simulink model "Plant"  (R2018b)
settings: configuration reference "plant_config" (kept outside this file)
values from neighbouring files (symbols this model uses):
  PLANT_EXPORT = Simulink.Parameter(PLANT_EXPORT_VALUE)    [plant_model_init.m]
  PLANT_PARAM = Simulink.Parameter(PLANT_PARAM_VALUE)    [plant_model_init.m]
undefined symbols (not defined in the file or in its folder): acc_x, acc_x_O, acc_y, acc_y_O, acc_z, acc_z_O, alt, alt_0, day, DiscIntNeverNeededParam, fixType, flags, gSpeed, gyr_x, gyr_y, gyr_z, h_R, hAcc, heading, headingAcc, height, hMSL, hour, iTOW, lat, lon, M_BO, M_OB, mag_x, mag_y, mag_z, month, nano, numSV, pDOP, phi, PLANT_CONST, plant_model, pressure, prop_vel, psi, quat, reserved1, reserved2, rot_x_B, rot_y_B, rot_z_B, sAcc, sec, Sensor_Model, tAcc, temperature, temprature, theta, timestamp, vAcc, valid, vel_x_O, vel_y_O, vel_z_O ... (+6)
libraries: FMT_Model_Lib x13, dspsrcs4 x6, simulink x4, aerolibatmos2 x1
(part 1 of 2)
settings Model: Creator=jc  LastModifiedBy=zouji
settings ConfigSetRef: SourceLocation=Base Workspace

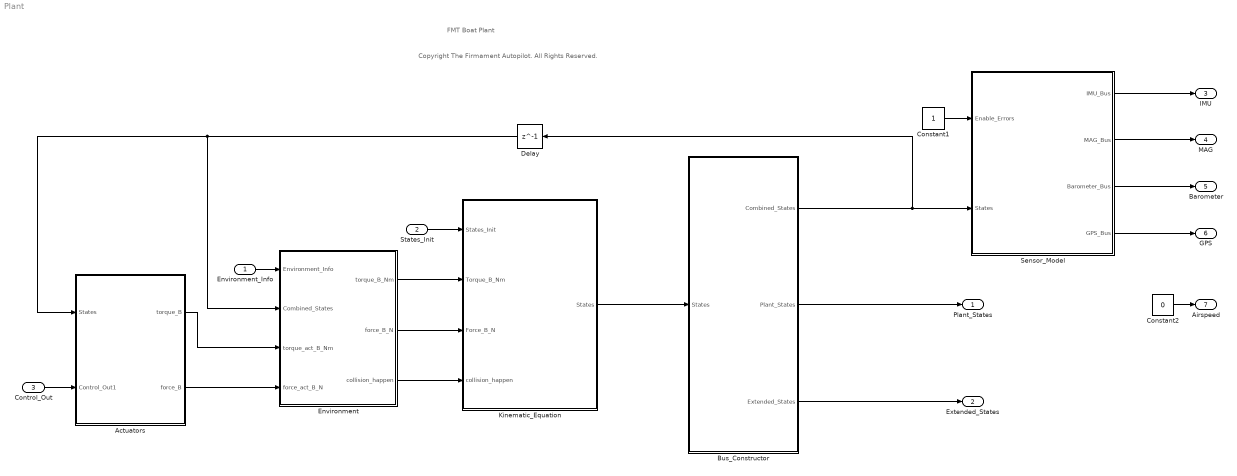
== system Plant ==
  note: FMT Boat Plant
  note: Copyright The Firmament Autopilot. All Rights Reserved.
  Environment_Info : Inport  OutDataTypeStr=Bus: Environment_Info_Bus  Interpolate=off
  States_Init : Inport  Port=2  OutDataTypeStr=Bus: States_Init_Bus  Interpolate=off
  Control_Out : Inport  Port=3  OutDataTypeStr=Bus: Control_Out_Bus  Interpolate=off
  Actuators : Subsystem  TreatAsAtomicUnit=on
  Bus_Constructor : Subsystem  TreatAsAtomicUnit=on  mask{lat_0=PLANT_PARAM.LAT_0, lon_0=PLANT_PARAM.LON_0, hgt_0=PLANT_PARAM.ALT_0}
      mask prompts: lat_0 "init latitude (rad)"; lon_0 "init lontitude (rad)"; hgt_0 "init height (m)"
  Constant1 : Constant  OutDataTypeStr=Inherit: Inherit via back propagation
  Constant2 : Constant  Value=0  OutDataTypeStr=Bus: AirSpeed_Bus
  Delay : Delay  DelayLength=1
  Environment : Subsystem  TreatAsAtomicUnit=on
  Kinematic_Equation : Subsystem  TreatAsAtomicUnit=on
  Sensor_Model : Subsystem  TreatAsAtomicUnit=on
  Plant_States : Outport  OutDataTypeStr=Bus: Plant_States_Bus
  Extended_States : Outport  Port=2  OutDataTypeStr=Bus: Extended_States_Bus
  IMU : Outport  Port=3  OutDataTypeStr=Bus: IMU_Bus
  MAG : Outport  Port=4  OutDataTypeStr=Bus: MAG_Bus
  Barometer : Outport  Port=5  OutDataTypeStr=Bus: Barometer_Bus
  GPS : Outport  Port=6  OutDataTypeStr=Bus: GPS_uBlox_Bus
  Airspeed : Outport  Port=7  OutDataTypeStr=Bus: AirSpeed_Bus
  wires:
  Kinematic_Equation/1(States) -> Bus_Constructor/1(States)
  Control_Out/1 -> Actuators/2(Control_Out1)
  Constant1/1 -> Sensor_Model/1(Enable_Errors)
  Sensor_Model/1(IMU_Bus) -> IMU/1
  Sensor_Model/2(MAG_Bus) -> MAG/1
  Sensor_Model/3(Barometer_Bus) -> Barometer/1
  Sensor_Model/4(GPS_Bus) -> GPS/1
  Bus_Constructor/3(Extended_States) -> Extended_States/1
  Bus_Constructor/1(Combined_States) -> Sensor_Model/2(States), Delay/1
  Constant2/1 -> Airspeed/1
  Bus_Constructor/2(Plant_States) -> Plant_States/1
  Delay/1 -> Environment/2(Combined_States), Actuators/1(States)
  Environment/3(collision_happen) -> Kinematic_Equation/4(collision_happen)
  States_Init/1 -> Kinematic_Equation/1(States_Init)
  Actuators/2(force_B) -> Environment/4(force_act_B_N)
  Actuators/1(torque_B) -> Environment/3(torque_act_B_Nm)
  Environment_Info/1 -> Environment/1(Environment_Info)
  Environment/1(torque_B_Nm) -> Kinematic_Equation/2(Torque_B_Nm)
  Environment/2(force_B_N) -> Kinematic_Equation/3(Force_B_N)

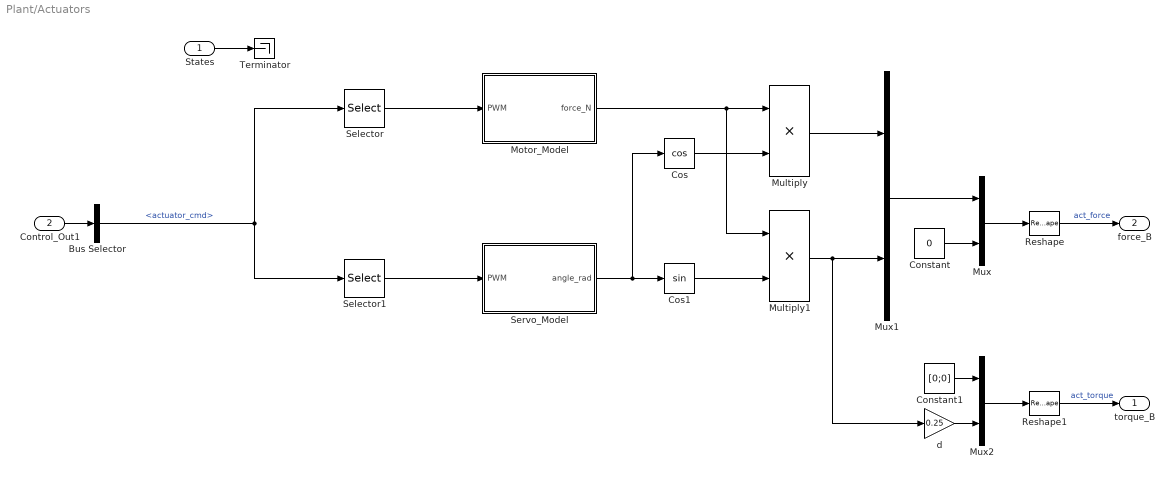
== system Plant/Actuators ==
  States : Inport
  Control_Out1 : Inport  Port=2
  Bus Selector : BusSelector  OutputSignals=actuator_cmd
  Constant : Constant  Value=0  OutDataTypeStr=single
  Constant1 : Constant  Value=[0;0]  VectorParams1D=off  OutDataTypeStr=single
  Cos : Trigonometry  Operator=cos
  Cos1 : Trigonometry
  Motor_Model : Subsystem
  Multiply : Product
  Multiply1 : Product
  Mux : Mux  Inputs=2
  Mux1 : Mux  Inputs=2
  Mux2 : Mux  Inputs=2
  Reshape : Reshape  OutputDimensionality=Column vector (2-D)
  Reshape1 : Reshape  OutputDimensionality=Column vector (2-D)
  Selector : Selector  InputPortWidth=16  IndexOptions=Index vector (dialog)  Indices=1  OutputSizes=1
  Selector1 : Selector  InputPortWidth=16  IndexOptions=Index vector (dialog)  Indices=2  OutputSizes=1
  Servo_Model : Subsystem
  Terminator : Terminator
  d : Gain  Gain=0.25
  torque_B : Outport
  force_B : Outport  Port=2
  wires:
  Control_Out1/1 -> Bus Selector/1
  States/1 -> Terminator/1
  Selector/1 -> Motor_Model/1(PWM)
  Selector1/1 -> Servo_Model/1(PWM)
  Bus Selector/1 -> Selector1/1, Selector/1  "<actuator_cmd>"
  Servo_Model/1(angle_rad) -> Cos1/1, Cos/1
  Cos/1 -> Multiply/2
  Motor_Model/1(force_N) -> Multiply1/1, Multiply/1
  Cos1/1 -> Multiply1/2
  Multiply/1 -> Mux1/1
  Constant/1 -> Mux/2
  Mux1/1 -> Mux/1
  Mux/1 -> Reshape/1
  Reshape/1 -> force_B/1  "act_force"
  Multiply1/1 -> d/1, Mux1/2
  Mux2/1 -> Reshape1/1
  Reshape1/1 -> torque_B/1  "act_torque"
  Constant1/1 -> Mux2/1
  d/1 -> Mux2/2

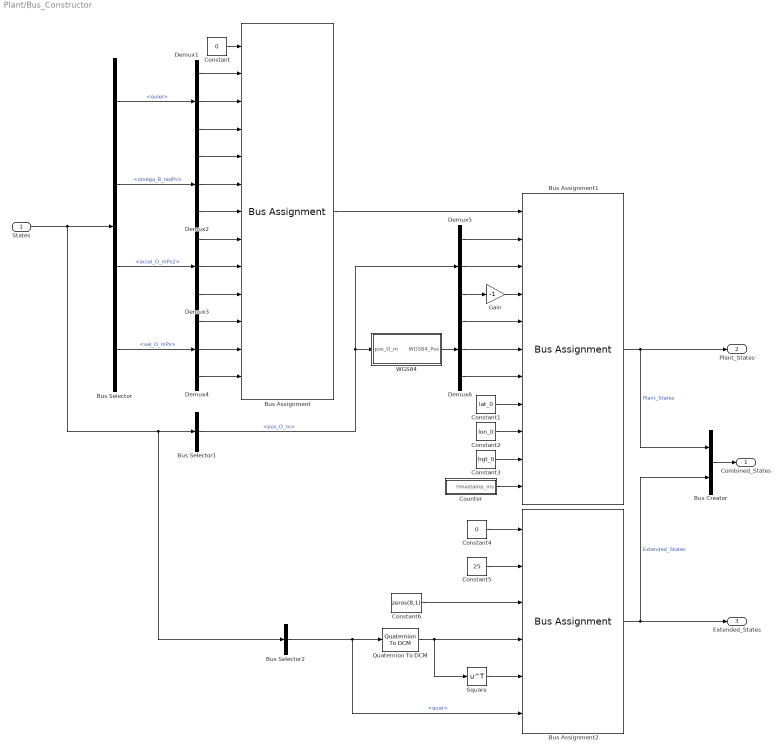
== system Plant/Bus_Constructor ==
  States : Inport
  Bus Assignment : BusAssignment  AssignedSignals=phi,theta,psi,rot_x_B,rot_y_B,rot_z_B,acc_x_O,acc_y_O,acc_z_O,vel_x_O,vel_y_O,vel_z_O
  Bus Assignment1 : BusAssignment  AssignedSignals=x_R,y_R,h_R,lat,lon,alt,lat_0,lon_0,alt_0,timestamp
  Bus Assignment2 : BusAssignment  AssignedSignals=temprature,prop_vel,M_BO,M_OB,quat
  Bus Creator : BusCreator  Inputs=2
  Bus Selector : BusSelector  OutputSignals=euler,omega_B_radPs,accel_O_mPs2,vel_O_mPs
  Bus Selector1 : BusSelector  OutputSignals=pos_O_m
  Bus Selector2 : BusSelector  OutputSignals=quat
  Constant : Constant  Value=0  OutDataTypeStr=Bus: Plant_States_Bus
  Constant1 : Constant  Value=lat_0
  Constant2 : Constant  Value=lon_0
  Constant3 : Constant  Value=hgt_0
  Constant4 : Constant  Value=0  OutDataTypeStr=Bus: Extended_States_Bus
  Constant5 : Constant  Value=25  OutDataTypeStr=Inherit: Inherit via back propagation
  Constant6 : Constant  Value=zeros(8,1)  OutDataTypeStr=single
  Counter : Subsystem
  Demux{1..6} (6 alike) : Demux  Outputs=3
  Gain : Gain  Gain=-1  OutDataTypeStr=Inherit: Same as input
  Quaternion To DCM : FMT_Model_Lib/Quaternion/Quaternion To DCM
      settings: SourceProductName=FMT Toolbox
  Square : Math  Operator=transpose  SaturateOnIntegerOverflow=on
  WGS84 : Subsystem
  Combined_States : Outport
  Plant_States : Outport  Port=2
  Extended_States : Outport  Port=3
  wires:
  Constant/1 -> Bus Assignment/1
  States/1 -> Bus Selector2/1, Bus Selector1/1, Bus Selector/1
  Bus Selector/1 -> Demux1/1  "<euler>"
  Bus Selector/2 -> Demux2/1  "<omega_B_radPs>"
  Bus Selector/3 -> Demux3/1  "<accel_O_mPs2>"
  Bus Selector/4 -> Demux4/1  "<vel_O_mPs>"
  Bus Assignment/1 -> Bus Assignment1/1
  Bus Selector1/1 -> Demux5/1, WGS84/1(pos_O_m)  "<pos_O_m>"
  Bus Assignment1/1 -> Plant_States/1, Bus Creator/1  "Plant_States"
  Demux1/2 -> Bus Assignment/3
  Demux5/3 -> Gain/1
  WGS84/1(WGS84_Pos) -> Demux6/1
  Demux1/1 -> Bus Assignment/2
  Demux1/3 -> Bus Assignment/4
  Demux2/1 -> Bus Assignment/5
  Demux2/2 -> Bus Assignment/6
  Demux2/3 -> Bus Assignment/7
  Demux3/1 -> Bus Assignment/8
  Demux3/2 -> Bus Assignment/9
  Demux3/3 -> Bus Assignment/10
  Demux4/1 -> Bus Assignment/11
  Demux4/2 -> Bus Assignment/12
  Demux4/3 -> Bus Assignment/13
  Demux5/2 -> Bus Assignment1/3
  Gain/1 -> Bus Assignment1/4
  Demux5/1 -> Bus Assignment1/2
  Demux6/1 -> Bus Assignment1/5
  Demux6/2 -> Bus Assignment1/6
  Demux6/3 -> Bus Assignment1/7
  Constant2/1 -> Bus Assignment1/9
  Constant1/1 -> Bus Assignment1/8
  Constant3/1 -> Bus Assignment1/10
  Constant4/1 -> Bus Assignment2/1
  Constant5/1 -> Bus Assignment2/2
  Constant6/1 -> Bus Assignment2/3
  Bus Selector2/1 -> Quaternion To DCM/1, Bus Assignment2/6  "<quat>"
  Bus Assignment2/1 -> Bus Creator/2, Extended_States/1  "Extended_States"
  Bus Creator/1 -> Combined_States/1
  Counter/1(timestamp_ms) -> Bus Assignment1/11
  Square/1 -> Bus Assignment2/5
  Quaternion To DCM/1 -> Square/1, Bus Assignment2/4

== system Plant/Environment ==
  Environment_Info : Inport
  Combined_States : Inport  Port=2
  torque_act_B_Nm : Inport  Port=3
  force_act_B_N : Inport  Port=4
  Constant : Constant  Value=0  OutDataTypeStr=Inherit: Inherit via back propagation
  Sum : Sum  Inputs=|++
  Sum1 : Sum  Inputs=|++
  Terminator : Terminator
  Water_Drag : Subsystem  mask{xu=1, xuu=0.5, yv=10, yvv=5, nr=4, nrr=1, mass=plant_model.mass, izz=plant_model.Jzz}
  torque_B_Nm : Outport
  force_B_N : Outport  Port=2
  collision_happen : Outport  Port=3
  wires:
  Environment_Info/1 -> Terminator/1
  Constant/1 -> collision_happen/1
  Combined_States/1 -> Water_Drag/1(Combined_States)
  Water_Drag/1(torque_B_Nm) -> Sum/1  "water_torque"
  Sum/1 -> torque_B_Nm/1  "torque_B_Nm"
  torque_act_B_Nm/1 -> Sum/2
  Water_Drag/2(force_B_N) -> Sum1/1  "water_force"
  force_act_B_N/1 -> Sum1/2
  Sum1/1 -> force_B_N/1  "force_B_N"

== system Plant/Kinematic_Equation ==
  States_Init : Inport
  Torque_B_Nm : Inport  Port=2
  Force_B_N : Inport  Port=3
  collision_happen : Inport  Port=4
  Attitude_Dynamic : Subsystem  mask{Ixx=plant_model.Jxx, Iyy=plant_model.Jyy, Izz=plant_model.Jzz}
  Bus Creator : BusCreator  Inputs=7
  Constant : Constant  Value=0  OutDataTypeStr=Inherit: Inherit via back propagation
  Position_Dynamic : Subsystem  mask{mass=plant_model.mass}
  States : Outport
  wires:
  Attitude_Dynamic/2(omega_B_radPs) -> Position_Dynamic/2(omega_B_radPs), Bus Creator/2  "omega_B_radPs"
  Attitude_Dynamic/3(quat) -> Position_Dynamic/3(quat), Bus Creator/3  "quat"
  collision_happen/1 -> Position_Dynamic/4(vel_reset)
  Bus Creator/1 -> States/1  "states"
  Attitude_Dynamic/1(dot_omega_B_radPs2) -> Bus Creator/1  "dot_omega_B_radPs2"
  Attitude_Dynamic/4(euler) -> Bus Creator/4  "euler"
  Position_Dynamic/1(accel_O_mPs2) -> Bus Creator/5  "accel_O_mPs2"
  Position_Dynamic/2(vel_O_mPs) -> Bus Creator/6  "vel_O_mPs"
  Position_Dynamic/3(pos_O_m) -> Bus Creator/7  "pos_O_m"
  Force_B_N/1 -> Position_Dynamic/1(force_B_N)
  Torque_B_Nm/1 -> Attitude_Dynamic/1(torque_B_Nm)
  Constant/1 -> Attitude_Dynamic/2(rate_reset)
  States_Init/1 -> Position_Dynamic/5(States_Init), Attitude_Dynamic/3(States_Init)

== system Plant/Sensor_Model ==
  Enable_Errors : Inport  OutDataTypeStr=uint8
  States : Inport  Port=2
  Counter : Subsystem
  Sensor_Barometer : Subsystem  TreatAsAtomicUnit=on
  Sensor_GPS : Subsystem  TreatAsAtomicUnit=on
  Sensor_IMU : Subsystem  TreatAsAtomicUnit=on
  Sensor_MAG : Subsystem  TreatAsAtomicUnit=on
  IMU_Bus : Outport
  MAG_Bus : Outport  Port=2
  Barometer_Bus : Outport  Port=3
  GPS_Bus : Outport  Port=4
  wires:
  Counter/1(timestamp_ms) -> Sensor_Barometer/3(timestamp_ms), Sensor_MAG/3(timestamp_ms), Sensor_IMU/3(timestamp_ms), Sensor_GPS/3(timestamp_ms)
  States/1 -> Sensor_GPS/1(States), Sensor_Barometer/1(States), Sensor_MAG/1(States), Sensor_IMU/1(States)
  Sensor_Barometer/1(Barometer_Bus) -> Barometer_Bus/1
  Sensor_MAG/1(MAG_Bus) -> MAG_Bus/1
  Sensor_IMU/1(IMU_Bus) -> IMU_Bus/1
  Enable_Errors/1 -> Sensor_IMU/2(Enable_Errors), Sensor_GPS/2(Enable_Errors), Sensor_Barometer/2(Enable_Errors), Sensor_MAG/2(Enable_Errors)
  Sensor_GPS/1(GPS_Bus) -> GPS_Bus/1

== system Plant/Actuators/Motor_Model ==
  PWM : Inport
  Bias : Bias  Bias=-60.6
  Dead Zone : DeadZone  LowerValue=-1  UpperValue=1  SaturateOnIntegerOverflow=on
  Gain : Gain  Gain=0.0404  OutDataTypeStr=single
  force_N : Outport
  wires:
  Gain/1 -> Bias/1
  Dead Zone/1 -> force_N/1
  PWM/1 -> Gain/1
  Bias/1 -> Dead Zone/1

== system Plant/Actuators/Servo_Model ==
  PWM : Inport
  Bias : Bias  Bias=-270
  Dead Zone : DeadZone  LowerValue=-2  UpperValue=2  SaturateOnIntegerOverflow=on
  Deg2Rad : Gain  Gain=pi/180
  Gain : Gain  Gain=0.18  OutDataTypeStr=single
  Saturation : Saturate  UpperLimit=90  LowerLimit=-90
  angle_rad : Outport
  wires:
  PWM/1 -> Gain/1
  Bias/1 -> Dead Zone/1
  Gain/1 -> Bias/1
  Deg2Rad/1 -> angle_rad/1
  Dead Zone/1 -> Saturation/1
  Saturation/1 -> Deg2Rad/1

== system Plant/Bus_Constructor/Counter ==
  Data Type Conversion2 : DataTypeConversion  OutDataTypeStr=uint32
  Delay : Delay  DelayLength=1  InitialCondition=0
  Sum : Sum  Inputs=|++
  dt : Constant  Value=PLANT_EXPORT.period  OutDataTypeStr=uint32
  timestamp_ms : Outport
  wires:
  dt/1 -> Sum/1
  Sum/1 -> Delay/1
  Delay/1 -> Data Type Conversion2/1
  Data Type Conversion2/1 -> timestamp_ms/1, Sum/2

== system Plant/Bus_Constructor/WGS84 ==
  pos_O_m : Inport
  Add : Sum
  Constant1 : Constant  Value=lat_0
  Constant2 : Constant  Value=lon_0
  Constant3 : Constant  Value=hgt_0
  Data Type Conversion : DataTypeConversion  OutDataTypeStr=double
  Delay : Delay  DelayLength=1
  Delay1 : Delay  DelayLength=1  InitialConditionSource=Input port  InitialCondition=[lat_0;lon_0;hgt_0]
      settings: InputPortMap=u0,p4
  Demux : Demux  Outputs=3
  Divide : Product  Inputs=/*
  Mux : Mux  Inputs=3
  Mux1 : Mux  Inputs=3
  Subtract : Sum  Inputs=+-
  Terminator : Terminator
  WGS84_Derivative : Subsystem
  Zero_Value_Exclusion : Subsystem
  WGS84_Pos : Outport
  wires:
  pos_O_m/1 -> Data Type Conversion/1
  Delay/1 -> Subtract/2
  WGS84_Derivative/1(dx_dlat) -> Mux/1
  Mux/1 -> Zero_Value_Exclusion/1(u)
  Zero_Value_Exclusion/1(y) -> Divide/1
  WGS84_Derivative/3(dz_dh) -> Mux/3
  WGS84_Derivative/2(dy_dlon) -> Mux/2
  Subtract/1 -> Divide/2
  Divide/1 -> Add/1
  Delay1/1 -> Add/2, Demux/1
  Add/1 -> Delay1/1, WGS84_Pos/1
  Demux/1 -> WGS84_Derivative/1(lat_0)
  Demux/3 -> WGS84_Derivative/2(h_0)
  Demux/2 -> Terminator/1
  Data Type Conversion/1 -> Delay/1, Subtract/1
  Mux1/1 -> Delay1/2
  Constant2/1 -> Mux1/2
  Constant1/1 -> Mux1/1
  Constant3/1 -> Mux1/3

== system Plant/Environment/Water_Drag ==
  Combined_States : Inport
  Bus Selector : BusSelector  OutputSignals=Extended_States.M_BO,Plant_States.vel_x_O,Plant_States.vel_y_O,Plant_States.vel_z_O
  Bus Selector1 : BusSelector  OutputSignals=Plant_States.rot_z_B
  Multiply : Product  Multiplication=Matrix(*)
  Mux : Mux  Inputs=3
  Water_Force : Subsystem
  Water_Torque : Subsystem
  torque_B_Nm : Outport
  force_B_N : Outport  Port=2
  wires:
  Combined_States/1 -> Bus Selector/1, Bus Selector1/1
  Bus Selector/2 -> Mux/1  "<vel_x_O>"
  Bus Selector/3 -> Mux/2  "<vel_y_O>"
  Bus Selector/4 -> Mux/3  "<vel_z_O>"
  Mux/1 -> Multiply/2
  Bus Selector/1 -> Multiply/1  "<M_BO>"
  Multiply/1 -> Water_Torque/1(vel_B), Water_Force/1(vel_B)
  Bus Selector1/1 -> Water_Force/2(r), Water_Torque/2(r)  "<rot_z_B>"
  Water_Torque/1(torque_B_Nm) -> torque_B_Nm/1
  Water_Force/1(force_B_N) -> force_B_N/1

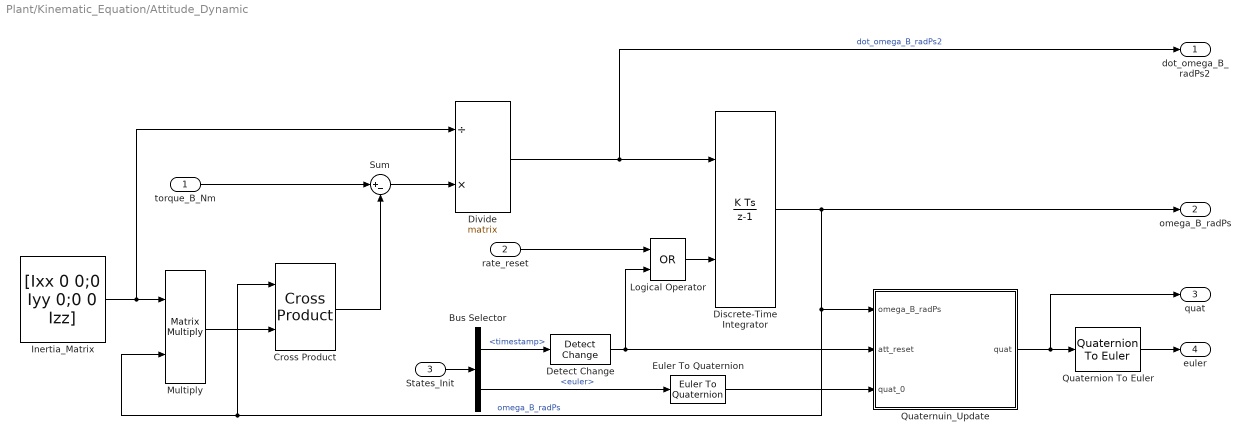
== system Plant/Kinematic_Equation/Attitude_Dynamic ==
  torque_B_Nm : Inport
  rate_reset : Inport  Port=2
  States_Init : Inport  Port=3
  Bus Selector : BusSelector  OutputSignals=timestamp,euler
  Cross Product : FMT_Model_Lib/Math/Cross Product
      settings: SourceProductName=FMT Toolbox
  Detect Change : simulink/Logic and Bit Operations/Detect Change  vinit=0  OutDataTypeStr=boolean
  Discrete-Time Integrator : DiscreteIntegrator  ExternalReset=level  InitialCondition=[0;0;0]  SampleTime=-1  ICPrevOutput=DiscIntNeverNeededParam  ICPrevScaledInput=DiscIntNeverNeededParam
  Divide : Product  Inputs=/*  Multiplication=Matrix(*)  OutDataTypeStr=Inherit: Same as first input
  Euler To Quaternion : FMT_Model_Lib/Quaternion/Euler To Quaternion
      settings: SourceProductName=FMT Toolbox
  Inertia_Matrix : Constant  Value=[Ixx 0 0;0 Iyy 0;0 0 Izz]  OutDataTypeStr=single
  Logical Operator : Logic  Operator=OR  AllPortsSameDT=off  OutDataTypeStr=boolean
  Multiply : Product  Multiplication=Matrix(*)  OutDataTypeStr=Inherit: Same as first input
  Quaternion To Euler : FMT_Model_Lib/Quaternion/Quaternion To Euler
      settings: SourceProductName=FMT Toolbox
  Quaternuin_Update : Subsystem
  Sum : Sum  Inputs=|+-  OutDataTypeStr=Inherit: Same as first input
  dot_omega_B_radPs2 : Outport
  omega_B_radPs : Outport  Port=2
  quat : Outport  Port=3
  euler : Outport  Port=4
  wires:
  Quaternion To Euler/1 -> euler/1
  Quaternuin_Update/1(quat) -> Quaternion To Euler/1, quat/1
  rate_reset/1 -> Logical Operator/1
  Divide/1 -> dot_omega_B_radPs2/1, Discrete-Time Integrator/1  "dot_omega_B_radPs2"
  Sum/1 -> Divide/2
  Cross Product/1 -> Sum/2
  torque_B_Nm/1 -> Sum/1
  Multiply/1 -> Cross Product/2
  Inertia_Matrix/1 -> Multiply/1, Divide/1
  Discrete-Time Integrator/1 -> omega_B_radPs/1, Cross Product/1, Multiply/2, Quaternuin_Update/1(omega_B_radPs)  "omega_B_radPs"
  States_Init/1 -> Bus Selector/1
  Bus Selector/1 -> Detect Change/1  "<timestamp>"
  Logical Operator/1 -> Discrete-Time Integrator/2
  Detect Change/1 -> Quaternuin_Update/2(att_reset), Logical Operator/2
  Bus Selector/2 -> Euler To Quaternion/1  "<euler>"
  Euler To Quaternion/1 -> Quaternuin_Update/3(quat_0)

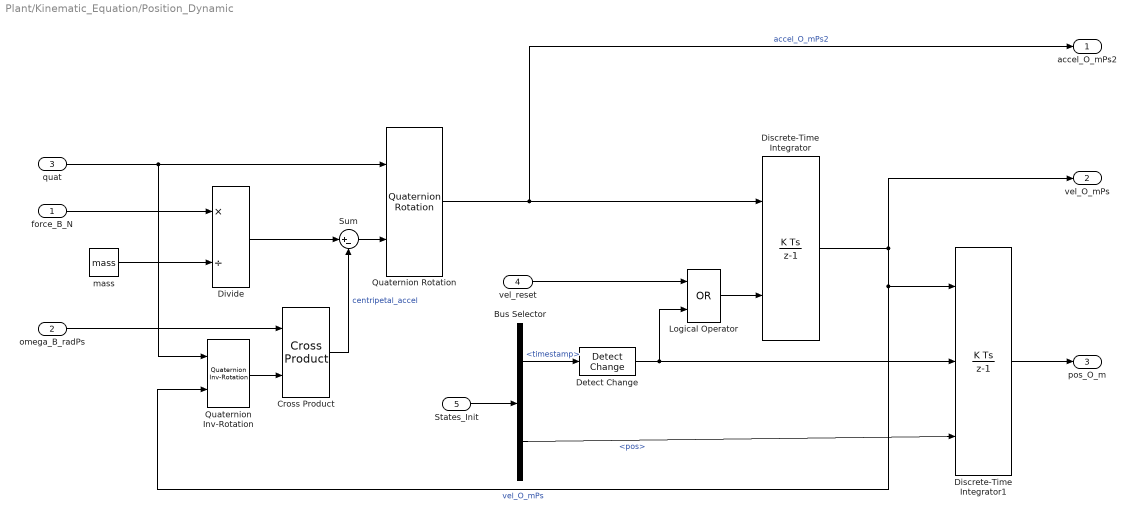
== system Plant/Kinematic_Equation/Position_Dynamic ==
  force_B_N : Inport
  omega_B_radPs : Inport  Port=2
  quat : Inport  Port=3
  vel_reset : Inport  Port=4
  States_Init : Inport  Port=5
  Bus Selector : BusSelector  OutputSignals=timestamp,pos
  Cross Product : FMT_Model_Lib/Math/Cross Product
      settings: SourceProductName=FMT Toolbox
  Detect Change : simulink/Logic and Bit Operations/Detect Change  vinit=0  OutDataTypeStr=boolean
  Discrete-Time Integrator : DiscreteIntegrator  ExternalReset=level  InitialCondition=[0;0;0]  SampleTime=-1  ICPrevOutput=DiscIntNeverNeededParam  ICPrevScaledInput=DiscIntNeverNeededParam
  Discrete-Time Integrator1 : DiscreteIntegrator  ExternalReset=level  InitialConditionSource=external  InitialCondition=[0;0;0]  SampleTime=-1  ICPrevOutput=DiscIntNeverNeededParam  ICPrevScaledInput=DiscIntNeverNeededParam
  Divide : Product  Inputs=*/
  Logical Operator : Logic  Operator=OR  AllPortsSameDT=off  OutDataTypeStr=boolean
  Quaternion Inv-Rotation : FMT_Model_Lib/Quaternion/Quaternion Inv-Rotation
      settings: SourceProductName=FMT Toolbox
  Quaternion Rotation : FMT_Model_Lib/Quaternion/Quaternion Rotation
      settings: SourceProductName=FMT Toolbox
  Sum : Sum  Inputs=|+-
  mass : Constant  Value=mass  OutDataTypeStr=single
  accel_O_mPs2 : Outport
  vel_O_mPs : Outport  Port=2
  pos_O_m : Outport  Port=3
  wires:
  force_B_N/1 -> Divide/1
  mass/1 -> Divide/2
  Discrete-Time Integrator/1 -> Quaternion Inv-Rotation/2, Discrete-Time Integrator1/1, vel_O_mPs/1  "vel_O_mPs"
  Divide/1 -> Sum/1
  Cross Product/1 -> Sum/2  "centripetal_accel"
  Sum/1 -> Quaternion Rotation/2
  quat/1 -> Quaternion Inv-Rotation/1, Quaternion Rotation/1
  Discrete-Time Integrator1/1 -> pos_O_m/1
  Quaternion Rotation/1 -> accel_O_mPs2/1, Discrete-Time Integrator/1  "accel_O_mPs2"
  Quaternion Inv-Rotation/1 -> Cross Product/2
  omega_B_radPs/1 -> Cross Product/1
  Logical Operator/1 -> Discrete-Time Integrator/2
  vel_reset/1 -> Logical Operator/1
  States_Init/1 -> Bus Selector/1
  Bus Selector/1 -> Detect Change/1  "<timestamp>"
  Detect Change/1 -> Discrete-Time Integrator1/2, Logical Operator/2
  Bus Selector/2 -> Discrete-Time Integrator1/3  "<pos>"

== system Plant/Sensor_Model/Counter ==
  Data Type Conversion2 : DataTypeConversion  OutDataTypeStr=uint32
  Memory1 : Memory
  Sum : Sum  Inputs=|++
  dt : Constant  Value=PLANT_EXPORT.period  OutDataTypeStr=uint32
  timestamp_ms : Outport
  wires:
  dt/1 -> Sum/1
  Sum/1 -> Memory1/1
  Memory1/1 -> Sum/2, Data Type Conversion2/1
  Data Type Conversion2/1 -> timestamp_ms/1

== system Plant/Sensor_Model/Sensor_Barometer ==
  States : Inport
  Enable_Errors : Inport  Port=2
  timestamp_ms : Inport  Port=3
  Barometer : Subsystem
  Bus_Constructor : Subsystem
  Barometer_Bus : Outport
  wires:
  Bus_Constructor/1(Barometer_Bus) -> Barometer_Bus/1
  timestamp_ms/1 -> Bus_Constructor/3(timestamp_ms)
  Enable_Errors/1 -> Barometer/1(Enable_Errors)
  States/1 -> Barometer/2(States)
  Barometer/1(pressure_Pa) -> Bus_Constructor/1(pressure_Pa)
  Barometer/2(temprature_K) -> Bus_Constructor/2(temperature_K)

== system Plant/Sensor_Model/Sensor_GPS ==
  States : Inport
  Enable_Errors : Inport  Port=2
  timestamp_ms : Inport  Port=3
  Bus_Constructor : Subsystem
  GPS : Subsystem
  GPS_Bus : Outport
  wires:
  Bus_Constructor/1(GPS_Bus) -> GPS_Bus/1
  timestamp_ms/1 -> Bus_Constructor/2(timestamp_ms)
  Enable_Errors/1 -> GPS/1(Enable_Errors)
  States/1 -> GPS/2(States)
  GPS/1(GPS_Raw) -> Bus_Constructor/1(GPS_Raw)

== system Plant/Sensor_Model/Sensor_IMU ==
  States : Inport
  Enable_Errors : Inport  Port=2
  timestamp_ms : Inport  Port=3
  Accelerometer : Subsystem
  Bus_Constructor : Subsystem
  Gyroscope : Subsystem
  IMU_Bus : Outport
  wires:
  Gyroscope/1(Gyro_Raw) -> Bus_Constructor/1(Gyro_Raw)
  Bus_Constructor/1(IMU_Bus) -> IMU_Bus/1
  States/1 -> Gyroscope/1(States), Accelerometer/1(States)
  Enable_Errors/1 -> Gyroscope/2(Enable_Errors), Accelerometer/2(Enable_Errors)
  Accelerometer/1(Acc_Raw) -> Bus_Constructor/2(Acc_Raw)
  timestamp_ms/1 -> Bus_Constructor/3(timestamp_ms)

== system Plant/Sensor_Model/Sensor_MAG ==
  States : Inport
  Enable_Errors : Inport  Port=2
  timestamp_ms : Inport  Port=3
  Bus_Constructor : Subsystem
  Magnetometer : Subsystem
  MAG_Bus : Outport
  wires:
  Magnetometer/1(Mag_Raw) -> Bus_Constructor/1(Mag_Raw)
  Bus_Constructor/1(MAG_Bus) -> MAG_Bus/1
  States/1 -> Magnetometer/1(States)
  Enable_Errors/1 -> Magnetometer/2(Enable_Errors)
  timestamp_ms/1 -> Bus_Constructor/2(timestamp_ms)

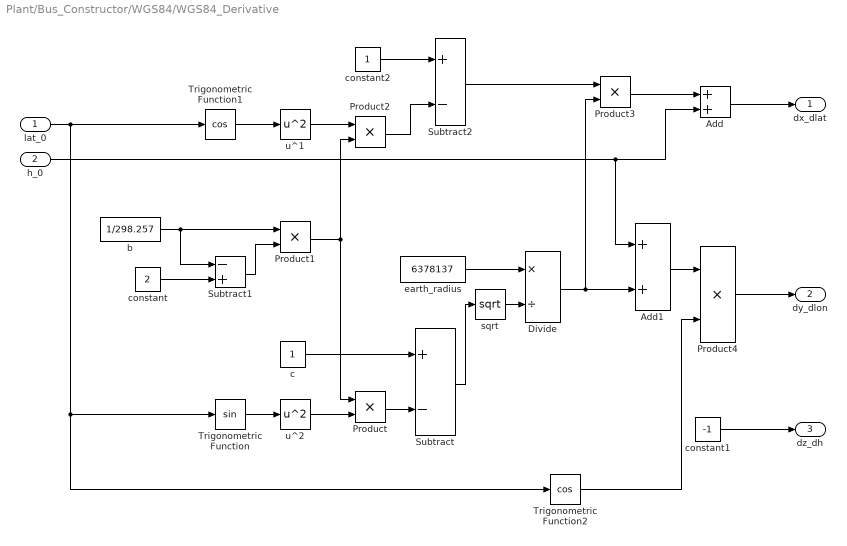
== system Plant/Bus_Constructor/WGS84/WGS84_Derivative ==
  lat_0 : Inport
  h_0 : Inport  Port=2
  Add : Sum
  Add1 : Sum
  Divide : Product  Inputs=*/
  Product{,1..4} (5 alike) : Product  RndMeth=Zero
  Subtract : Sum  Inputs=+-
  Subtract1 : Sum  Inputs=-+
  Subtract2 : Sum  Inputs=+-
  Trigonometric Function : Trigonometry
  Trigonometric Function1 : Trigonometry  Operator=cos
  Trigonometric Function2 : Trigonometry  Operator=cos
  b : Constant  Value=1/298.257
  c : Constant
  constant : Constant  Value=2
  constant1 : Constant  Value=-1
  constant2 : Constant
  earth_radius : Constant  Value=6378137
  sqrt : Math  Operator=sqrt  SaturateOnIntegerOverflow=on
  u^1 : Math  Operator=square  SaturateOnIntegerOverflow=on
  u^2 : Math  Operator=square  SaturateOnIntegerOverflow=on
  dx_dlat : Outport
  dy_dlon : Outport  Port=2
  dz_dh : Outport  Port=3  InitialOutput=1
  wires:
  constant1/1 -> dz_dh/1
  Product4/1 -> dy_dlon/1
  Add1/1 -> Product4/1
  Trigonometric Function2/1 -> Product4/2
  Product3/1 -> Add/1
  Subtract2/1 -> Product3/1
  Product2/1 -> Subtract2/2
  u^1/1 -> Product2/1
  Trigonometric Function1/1 -> u^1/1
  constant2/1 -> Subtract2/1
  h_0/1 -> Add1/1, Add/2
  Add/1 -> dx_dlat/1
  Divide/1 -> Product3/2, Add1/2
  sqrt/1 -> Divide/2
  Product1/1 -> Product2/2, Product/1
  Subtract1/1 -> Product1/2
  constant/1 -> Subtract1/2
  b/1 -> Subtract1/1, Product1/1
  Product/1 -> Subtract/2
  Subtract/1 -> sqrt/1
  c/1 -> Subtract/1
  u^2/1 -> Product/2
  Trigonometric Function/1 -> u^2/1
  lat_0/1 -> Trigonometric Function2/1, Trigonometric Function/1, Trigonometric Function1/1
  earth_radius/1 -> Divide/1

== system Plant/Bus_Constructor/WGS84/Zero_Value_Exclusion ==
  u : Inport
  Abs : Abs
  Constant : Constant
  Product : Product  RndMeth=Zero
  Saturation : Saturate  UpperLimit=10e7  LowerLimit=1e-6  LinearizeAsGain=off
  Sign : Signum
  Switch : Switch  Criteria=u2 ~= 0
  y : Outport
  wires:
  u/1 -> Sign/1, Abs/1
  Abs/1 -> Saturation/1
  Saturation/1 -> Product/1
  Sign/1 -> Switch/2, Switch/1
  Product/1 -> y/1
  Switch/1 -> Product/2
  Constant/1 -> Switch/3

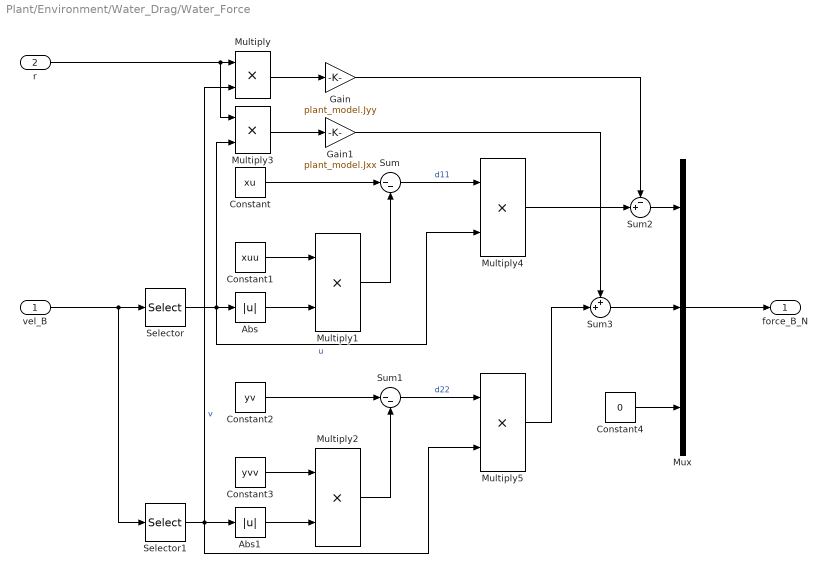
== system Plant/Environment/Water_Drag/Water_Force ==
  vel_B : Inport
  r : Inport  Port=2
  Abs : Abs
  Abs1 : Abs
  Constant : Constant  Value=xu  OutDataTypeStr=single
  Constant1 : Constant  Value=xuu  OutDataTypeStr=single
  Constant2 : Constant  Value=yv  OutDataTypeStr=single
  Constant3 : Constant  Value=yvv  OutDataTypeStr=single
  Constant4 : Constant  Value=0  OutDataTypeStr=single
  Gain : Gain  Gain=plant_model.Jyy
  Gain1 : Gain  Gain=plant_model.Jxx
  Multiply{,1..5} (6 alike) : Product
  Mux : Mux  Inputs=3
  Selector : Selector  InputPortWidth=3  IndexOptions=Index vector (dialog)  Indices=1  OutputSizes=1
  Selector1 : Selector  InputPortWidth=3  IndexOptions=Index vector (dialog)  Indices=2  OutputSizes=1
  Sum : Sum  Inputs=|--
  Sum1 : Sum  Inputs=|--
  Sum2 : Sum  Inputs=-+|
  Sum3 : Sum  Inputs=++|
  force_B_N : Outport
  wires:
  Abs/1 -> Multiply1/2
  Sum1/1 -> Multiply5/1  "d22"
  Constant/1 -> Sum/1
  vel_B/1 -> Selector1/1, Selector/1
  Constant3/1 -> Multiply2/1
  Constant2/1 -> Sum1/1
  Multiply1/1 -> Sum/2
  Constant1/1 -> Multiply1/1
  Selector/1 -> Abs/1, Multiply3/2, Multiply4/2  "u"
  Selector1/1 -> Abs1/1, Multiply5/2, Multiply/2  "v"
  Sum/1 -> Multiply4/1  "d11"
  Abs1/1 -> Multiply2/2
  Multiply2/1 -> Sum1/2
  Multiply5/1 -> Sum3/2
  Constant4/1 -> Mux/3
  Mux/1 -> force_B_N/1
  r/1 -> Multiply3/1, Multiply/1
  Multiply/1 -> Gain/1
  Multiply4/1 -> Sum2/2
  Sum2/1 -> Mux/1
  Gain/1 -> Sum2/1
  Multiply3/1 -> Gain1/1
  Gain1/1 -> Sum3/1
  Sum3/1 -> Mux/2

== system Plant/Environment/Water_Drag/Water_Torque ==
  vel_B : Inport
  r : Inport  Port=2
  Abs2 : Abs
  Constant : Constant  Value=0  OutDataTypeStr=single
  Constant4 : Constant  Value=nr  OutDataTypeStr=single
  Constant5 : Constant  Value=nrr  OutDataTypeStr=single
  Gain : Gain  Gain=plant_model.Jxx-plant_model.Jyy
  Multiply : Product
  Multiply3 : Product
  Multiply6 : Product
  Mux : Mux  Inputs=3
  Selector : Selector  InputPortWidth=3  IndexOptions=Index vector (dialog)  Indices=1  OutputSizes=1
  Selector1 : Selector  InputPortWidth=3  IndexOptions=Index vector (dialog)  Indices=2  OutputSizes=1
  Sum : Sum  Inputs=-+|
  Sum2 : Sum  Inputs=|--
  torque_B_Nm : Outport
  wires:
  Abs2/1 -> Multiply3/2
  r/1 -> Multiply6/2, Abs2/1
  Sum2/1 -> Multiply6/1  "d33"
  Constant5/1 -> Multiply3/1
  Constant4/1 -> Sum2/1
  Multiply3/1 -> Sum2/2
  Constant/1 -> Mux/2, Mux/1
  Mux/1 -> torque_B_Nm/1
  vel_B/1 -> Selector/1, Selector1/1
  Selector/1 -> Multiply/1  "u"
  Selector1/1 -> Multiply/2  "v"
  Multiply/1 -> Gain/1
  Multiply6/1 -> Mux/3, Sum/2
  Gain/1 -> Sum/1

== system Plant/Kinematic_Equation/Attitude_Dynamic/Quaternuin_Update ==
  omega_B_radPs : Inport
  att_reset : Inport  Port=2
  quat_0 : Inport  Port=3
  Discrete-Time Integrator : DiscreteIntegrator  ExternalReset=level  InitialConditionSource=external  SampleTime=-1  ICPrevOutput=DiscIntNeverNeededParam  ICPrevScaledInput=DiscIntNeverNeededParam
  Gain : Gain  Gain=0.5  OutDataTypeStr=Inherit: Same as input
  Multiply : Product  Multiplication=Matrix(*)  OutDataTypeStr=Inherit: Same as first input
  Quaternion Normalize : FMT_Model_Lib/Quaternion/Quaternion Normalize
      settings: SourceProductName=FMT Toolbox
  Quaternion_Update_Maxtrix : Subsystem
  quat : Outport
  wires:
  Gain/1 -> Discrete-Time Integrator/1  "dot_q"
  Multiply/1 -> Gain/1
  Quaternion_Update_Maxtrix/1(W) -> Multiply/1
  omega_B_radPs/1 -> Quaternion_Update_Maxtrix/1(omega_B_radPs)
  Discrete-Time Integrator/1 -> quat/1, Multiply/2
  Quaternion Normalize/1 -> Discrete-Time Integrator/3
  att_reset/1 -> Discrete-Time Integrator/2
  quat_0/1 -> Quaternion Normalize/1

== system Plant/Sensor_Model/Sensor_Barometer/Barometer ==
  Enable_Errors : Inport
  States : Inport  Port=2
  Physical_Model : Subsystem
  Sensor_Model : Subsystem
  pressure_Pa : Outport
  temprature_K : Outport  Port=2
  wires:
  Physical_Model/1(Pressure_Pa) -> Sensor_Model/2(u)
  Enable_Errors/1 -> Sensor_Model/1(Enable_Errors)
  States/1 -> Physical_Model/1(States)
  Sensor_Model/1(y) -> pressure_Pa/1
  Physical_Model/2(Temperature_K) -> temprature_K/1

== system Plant/Sensor_Model/Sensor_Barometer/Bus_Constructor ==
  pressure_Pa : Inport  Unit=N/m^2
  temperature_K : Inport  Port=2  Unit=K
  timestamp_ms : Inport  Port=3
  Bus Assignment : BusAssignment  AssignedSignals=timestamp,pressure,temperature
  Constant : Constant  Value=0  OutDataTypeStr=Bus: Barometer_Bus
  Constant2 : Constant  Value=273.15
  Data Type Conversion : DataTypeConversion  OutDataTypeStr=single
  Data Type Conversion1 : DataTypeConversion  OutDataTypeStr=single
  Rate Transition : RateTransition  OutPortSampleTime=0.01
  Sum1 : Sum  Inputs=|+-
  Barometer_Bus : Outport
  wires:
  Data Type Conversion1/1 -> Bus Assignment/4
  Constant/1 -> Bus Assignment/1
  Data Type Conversion/1 -> Bus Assignment/3
  Bus Assignment/1 -> Rate Transition/1
  pressure_Pa/1 -> Data Type Conversion/1
  temperature_K/1 -> Sum1/1
  Rate Transition/1 -> Barometer_Bus/1
  Sum1/1 -> Data Type Conversion1/1
  Constant2/1 -> Sum1/2
  timestamp_ms/1 -> Bus Assignment/2

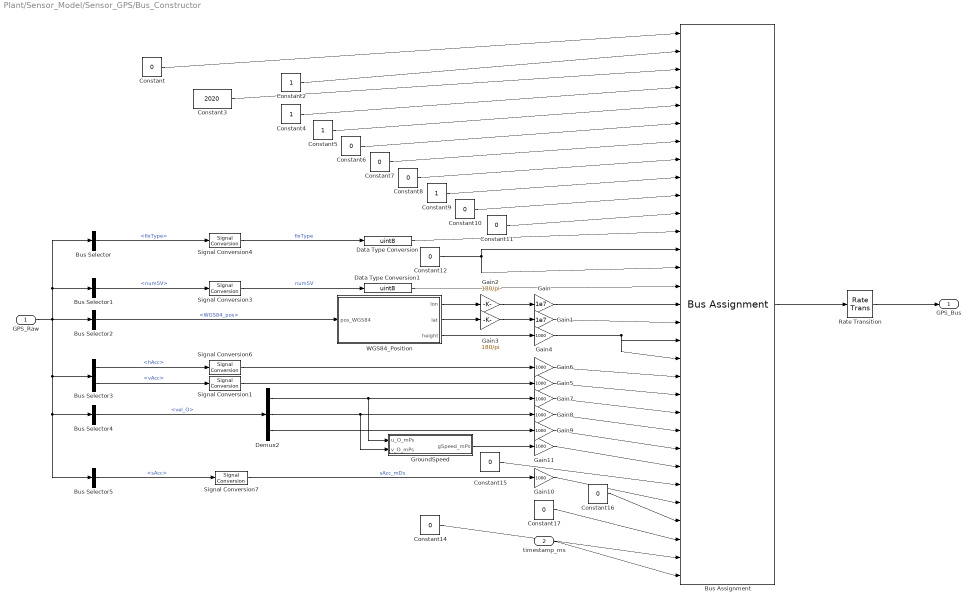
== system Plant/Sensor_Model/Sensor_GPS/Bus_Constructor ==
  GPS_Raw : Inport
  timestamp_ms : Inport  Port=2
  Bus Assignment : BusAssignment  AssignedSignals=iTOW,year,month,day,hour,min,sec,valid,tAcc,nano,fixType,flags,reserved1,numSV,lon,lat,height,hMSL,hAcc,vAcc,velN,velE,velD,gSpeed,heading,sAcc,headingAcc,pDOP,reserved2,timestamp
  Bus Selector : BusSelector  OutputSignals=fixType
  Bus Selector1 : BusSelector  OutputSignals=numSV
  Bus Selector2 : BusSelector  OutputSignals=WGS84_pos
  Bus Selector3 : BusSelector  OutputSignals=hAcc,vAcc
  Bus Selector4 : BusSelector  OutputSignals=vel_O
  Bus Selector5 : BusSelector  OutputSignals=sAcc
  Constant : Constant  Value=0  OutDataTypeStr=Bus: GPS_uBlox_Bus
  Constant10 : Constant  Value=0  OutDataTypeStr=uint32
  Constant11 : Constant  Value=0  OutDataTypeStr=int32
  Constant{6..8,12} (4 alike) : Constant  Value=0  OutDataTypeStr=uint8
  Constant14 : Constant  Value=0  OutDataTypeStr=uint16
  Constant15 : Constant  Value=0  OutDataTypeStr=int32
  Constant16 : Constant  Value=0  OutDataTypeStr=uint32
  Constant17 : Constant  Value=0  OutDataTypeStr=uint16
  Constant2 : Constant  OutDataTypeStr=uint32
  Constant3 : Constant  Value=2020  OutDataTypeStr=uint16
  Constant4 : Constant  OutDataTypeStr=uint8
  Constant5 : Constant  OutDataTypeStr=uint8
  Constant9 : Constant  OutDataTypeStr=uint8
  Data Type Conversion : DataTypeConversion  OutDataTypeStr=uint8
  Data Type Conversion1 : DataTypeConversion  OutDataTypeStr=uint8
  Demux2 : Demux  Outputs=3
  Gain : Gain  Gain=1e7  OutDataTypeStr=int32
      settings: AttributesFormatString=Gain: %<Gain>
  Gain1 : Gain  Gain=1e7  OutDataTypeStr=int32
      settings: AttributesFormatString=Gain: %<Gain>
  Gain10 : Gain  Gain=1000  OutDataTypeStr=uint32
      settings: AttributesFormatString=Gain: %<Gain>
  Gain{4,7..9,11} (5 alike) : Gain  Gain=1000  OutDataTypeStr=int32
      settings: AttributesFormatString=Gain: %<Gain>
  Gain2 : Gain  Gain=180/pi
      settings: AttributesFormatString=Gain: %<Gain>
  Gain3 : Gain  Gain=180/pi
      settings: AttributesFormatString=Gain: %<Gain>
  Gain5 : Gain  Gain=1000  OutDataTypeStr=uint32
      settings: AttributesFormatString=Gain: %<Gain>
  Gain6 : Gain  Gain=1000  OutDataTypeStr=uint32
      settings: AttributesFormatString=Gain: %<Gain>
  GroundSpeed : Subsystem
  Rate Transition : RateTransition  OutPortSampleTime=0.1
  Signal Conversion{1,3..4,6..7} (5 alike) : SignalConversion  OverrideOpt=off
  WGS84_Position : Subsystem
  GPS_Bus : Outport
  wires:
  Bus Selector5/1 -> Signal Conversion7/1  "<sAcc>"
  Bus Selector3/1 -> Signal Conversion6/1  "<hAcc>"
  Bus Selector1/1 -> Signal Conversion3/1  "<numSV>"
  Bus Selector4/1 -> Demux2/1  "<vel_O>"
  Gain5/1 -> Bus Assignment/21
  Constant15/1 -> Bus Assignment/26
  Data Type Conversion/1 -> Bus Assignment/12
  Constant17/1 -> Bus Assignment/29
  Gain4/1 -> Bus Assignment/19, Bus Assignment/18
  Constant16/1 -> Bus Assignment/28
  Gain3/1 -> Gain1/1
  Signal Conversion6/1 -> Gain6/1
  Gain6/1 -> Bus Assignment/20
  Gain11/1 -> Bus Assignment/25
  Gain8/1 -> Bus Assignment/23
  Gain7/1 -> Bus Assignment/22
  Gain10/1 -> Bus Assignment/27
  Constant/1 -> Bus Assignment/1
  Constant8/1 -> Bus Assignment/8
  Gain2/1 -> Gain/1
  Constant4/1 -> Bus Assignment/4
  Constant11/1 -> Bus Assignment/11
  Constant10/1 -> Bus Assignment/10
  Constant9/1 -> Bus Assignment/9
  Constant3/1 -> Bus Assignment/3
  Constant6/1 -> Bus Assignment/6
  Bus Assignment/1 -> Rate Transition/1
  Gain9/1 -> Bus Assignment/24
  Constant12/1 -> Bus Assignment/14, Bus Assignment/13
  Constant14/1 -> Bus Assignment/30
  GroundSpeed/1(gSpeed_mPs) -> Gain11/1
  Constant5/1 -> Bus Assignment/5
  Gain/1 -> Bus Assignment/16
  Data Type Conversion1/1 -> Bus Assignment/15
  Constant2/1 -> Bus Assignment/2
  Gain1/1 -> Bus Assignment/17
  Constant7/1 -> Bus Assignment/7
  Signal Conversion7/1 -> Gain10/1  "sAcc_mDs"
  Demux2/1 -> GroundSpeed/1(u_O_mPs), Gain7/1
  Demux2/2 -> Gain8/1, GroundSpeed/2(v_O_mPs)
  Demux2/3 -> Gain9/1
  Bus Selector2/1 -> WGS84_Position/1(pos_WGS84)  "<WGS84_pos>"
  WGS84_Position/1(lon) -> Gain2/1
  WGS84_Position/2(lat) -> Gain3/1
  WGS84_Position/3(height) -> Gain4/1
  Signal Conversion3/1 -> Data Type Conversion1/1  "numSV"
  Signal Conversion4/1 -> Data Type Conversion/1  "fixType"
  Bus Selector3/2 -> Signal Conversion1/1  "<vAcc>"
  Signal Conversion1/1 -> Gain5/1
  Rate Transition/1 -> GPS_Bus/1
  timestamp_ms/1 -> Bus Assignment/31
  GPS_Raw/1 -> Bus Selector3/1, Bus Selector4/1, Bus Selector5/1, Bus Selector2/1, Bus Selector1/1, Bus Selector/1
  Bus Selector/1 -> Signal Conversion4/1  "<fixType>"

== system Plant/Sensor_Model/Sensor_GPS/GPS ==
  Enable_Errors : Inport
  States : Inport  Port=2
  Bus_Constructor : Subsystem
  Physical_Model : Subsystem
  Sensor_Model : Subsystem
  GPS_Raw : Outport
  wires:
  Physical_Model/1(WGS84_pos_rad) -> Sensor_Model/2(WGS84_pos_rad)
  Physical_Model/2(vel_O_mPs) -> Sensor_Model/3(vel_O_mPs)
  States/1 -> Physical_Model/1(States)
  Enable_Errors/1 -> Sensor_Model/1(Enable_Errors)
  Sensor_Model/1(WGS84_pos_meas) -> Bus_Constructor/1(WGS84_pos_meas)
  Sensor_Model/2(vel_O_meas) -> Bus_Constructor/2(vel_O_meas)
  Sensor_Model/3(numSV) -> Bus_Constructor/3(numSV)
  Sensor_Model/4(fixType) -> Bus_Constructor/4(fixType)
  Sensor_Model/5(h_Acc_m) -> Bus_Constructor/5(h_Acc_m)
  Sensor_Model/6(v_Acc_m) -> Bus_Constructor/6(v_Acc_m)
  Sensor_Model/7(s_Acc_mDs) -> Bus_Constructor/7(s_Acc_mDs)
  Bus_Constructor/1(GPS_Raw) -> GPS_Raw/1

== system Plant/Sensor_Model/Sensor_IMU/Accelerometer ==
  States : Inport
  Enable_Errors : Inport  Port=2
  Bus_Constructor : Subsystem
  Physical_Model : Subsystem
  Sensor_Model : Subsystem
  Acc_Raw : Outport
  wires:
  Sensor_Model/1(y) -> Bus_Constructor/1(Output)
  States/1 -> Physical_Model/1(States)
  Physical_Model/1(sfor_B_mPs2) -> Sensor_Model/2(u)
  Bus_Constructor/1(Acc_Raw) -> Acc_Raw/1
  Enable_Errors/1 -> Physical_Model/2(Enable_Errors), Sensor_Model/1(Enable_Errors)

== system Plant/Sensor_Model/Sensor_IMU/Bus_Constructor ==
  Gyro_Raw : Inport
  Acc_Raw : Inport  Port=2
  timestamp_ms : Inport  Port=3
  Bus Assignment : BusAssignment  AssignedSignals=timestamp,gyr_x,gyr_y,gyr_z,acc_x,acc_y,acc_z
  Bus Selector : BusSelector  OutputSignals=Gyro_x_radPs,Gyro_y_radPs,Gyro_z_radPs
  Bus Selector1 : BusSelector  OutputSignals=Acc_x_mPs2,Acc_y_mPs2,Acc_z_mPs2
  Constant : Constant  Value=0  OutDataTypeStr=Bus: IMU_Bus
  IMU_Bus : Outport
  wires:
  Gyro_Raw/1 -> Bus Selector/1
  Acc_Raw/1 -> Bus Selector1/1
  Constant/1 -> Bus Assignment/1
  timestamp_ms/1 -> Bus Assignment/2
  Bus Assignment/1 -> IMU_Bus/1
  Bus Selector1/1 -> Bus Assignment/6  "<Acc_x_mPs2>"
  Bus Selector1/2 -> Bus Assignment/7  "<Acc_y_mPs2>"
  Bus Selector1/3 -> Bus Assignment/8  "<Acc_z_mPs2>"
  Bus Selector/1 -> Bus Assignment/3  "<Gyro_x_radPs>"
  Bus Selector/2 -> Bus Assignment/4  "<Gyro_y_radPs>"
  Bus Selector/3 -> Bus Assignment/5  "<Gyro_z_radPs>"

== system Plant/Sensor_Model/Sensor_IMU/Gyroscope ==
  States : Inport
  Enable_Errors : Inport  Port=2
  Bus_Constructor : Subsystem
  Physical_Model : Subsystem
  Sensor_Model : Subsystem
  Gyro_Raw : Outport
  wires:
  States/1 -> Physical_Model/1(States)
  Sensor_Model/1(y) -> Bus_Constructor/1(Output)
  Bus_Constructor/1(Gyro_Raw) -> Gyro_Raw/1
  Enable_Errors/1 -> Physical_Model/2(Enable_Errors), Sensor_Model/1(Enable_Errors)
  Physical_Model/1(gyr_B_radDs) -> Sensor_Model/2(u)

== system Plant/Sensor_Model/Sensor_MAG/Bus_Constructor ==
  Mag_Raw : Inport
  timestamp_ms : Inport  Port=2
  Bus Assignment : BusAssignment  AssignedSignals=timestamp,mag_x,mag_y,mag_z
  Bus Selector : BusSelector  OutputSignals=Mag_x_gauss,Mag_y_gauss,Mag_z_gauss
  Constant : Constant  Value=0  OutDataTypeStr=Bus: MAG_Bus
  Rate Transition : RateTransition  OutPortSampleTime=0.01
  MAG_Bus : Outport
  wires:
  Bus Assignment/1 -> Rate Transition/1
  Constant/1 -> Bus Assignment/1
  timestamp_ms/1 -> Bus Assignment/2
  Rate Transition/1 -> MAG_Bus/1
  Bus Selector/1 -> Bus Assignment/3  "<Mag_x_gauss>"
  Mag_Raw/1 -> Bus Selector/1
  Bus Selector/2 -> Bus Assignment/4  "<Mag_y_gauss>"
  Bus Selector/3 -> Bus Assignment/5  "<Mag_z_gauss>"

== system Plant/Sensor_Model/Sensor_MAG/Magnetometer ==
  States : Inport
  Enable_Errors : Inport  Port=2
  Bus_Constructor : Subsystem
  Physical_Model : Subsystem
  Sensor_Model : Subsystem
  Mag_Raw : Outport
  wires:
  Bus_Constructor/1(Mag_Raw) -> Mag_Raw/1
  Sensor_Model/1(y) -> Bus_Constructor/1(Output)
  States/1 -> Physical_Model/1(States)
  Physical_Model/1(mag_B_gauss) -> Sensor_Model/2(u)
  Enable_Errors/1 -> Sensor_Model/1(Enable_Errors)

== system Plant/Kinematic_Equation/Attitude_Dynamic/Quaternuin_Update/Quaternion_Update_Maxtrix ==
  omega_B_radPs : Inport
  Constant{,1..3} (4 alike) : Constant  Value=0  OutDataTypeStr=single
  Demux : Demux  Outputs=3
  Gain{1..4,6..7} (6 alike) : Gain  Gain=-1  OutDataTypeStr=Inherit: Same as input
  Matrix Concatenate{,1..3} (4 alike) : Concatenate  NumInputs=4
  Matrix Concatenate4 : Concatenate  NumInputs=4  Mode=Multidimensional array  ConcatenateDimension=2
  W : Outport
  wires:
  Gain1/1 -> Matrix Concatenate1/1
  Gain7/1 -> Matrix Concatenate3/2
  Matrix Concatenate2/1 -> Matrix Concatenate4/3  "col3"
  Constant2/1 -> Matrix Concatenate2/3
  Matrix Concatenate4/1 -> W/1
  Demux/1 -> Matrix Concatenate/2, Gain1/1, Gain4/1, Matrix Concatenate3/3  "w1"
  Matrix Concatenate/1 -> Matrix Concatenate4/1  "col1"
  Matrix Concatenate1/1 -> Matrix Concatenate4/2  "col2"
  Constant3/1 -> Matrix Concatenate3/4
  Gain6/1 -> Matrix Concatenate3/1
  Constant1/1 -> Matrix Concatenate1/2
  Matrix Concatenate3/1 -> Matrix Concatenate4/4  "col4"
  Demux/2 -> Matrix Concatenate1/4, Gain3/1, Gain7/1, Matrix Concatenate/3  "w2"
  Constant/1 -> Matrix Concatenate/1
  Gain3/1 -> Matrix Concatenate2/1
  Demux/3 -> Gain2/1, Matrix Concatenate2/2, Gain6/1, Matrix Concatenate/4  "w3"
  Gain2/1 -> Matrix Concatenate1/3
  omega_B_radPs/1 -> Demux/1
  Gain4/1 -> Matrix Concatenate2/4

== system Plant/Sensor_Model/Sensor_Barometer/Barometer/Physical_Model ==
  States : Inport
  Bus Selector1 : BusSelector  OutputSignals=Plant_States.alt
  Data Type Conversion : DataTypeConversion  OutDataTypeStr=single
  ISA Atmosphere Model : aerolibatmos2/ISA Atmosphere Model  custom=off  g=9.80665  gamma=1.4  R=287.0531  L=0.0065  h_trop=11000  h_strat=20000  rho0=1.225  P0=101325  T0=288.15  h0=0
      settings: SourceProductName=Aerospace Blockset
  Terminator : Terminator
  Terminator1 : Terminator
  Pressure_Pa : Outport
  Temperature_K : Outport  Port=2
  wires:
  States/1 -> Bus Selector1/1
  ISA Atmosphere Model/1 -> Temperature_K/1
  ISA Atmosphere Model/2 -> Terminator1/1
  ISA Atmosphere Model/4 -> Terminator/1
  Bus Selector1/1 -> Data Type Conversion/1  "<alt>"
  ISA Atmosphere Model/3 -> Pressure_Pa/1
  Data Type Conversion/1 -> ISA Atmosphere Model/1

== system Plant/Sensor_Model/Sensor_Barometer/Barometer/Sensor_Model ==
  Enable_Errors : Inport
  u : Inport  Port=2
  Add : Sum  InputSameDT=on  OutDataTypeStr=Inherit: Same as first input
  Saturation : Saturate  UpperLimit=Sensor_Model.Baro.Upper_limit  LowerLimit=Sensor_Model.Baro.Lower_limit  OutDataTypeStr=single
  Sensor_Error : Subsystem
  Sensor_Noise : Subsystem
  Switch : Switch  Criteria=u2 > Threshold
  y : Outport
  wires:
  Switch/1 -> y/1
  Saturation/1 -> Add/1
  Sensor_Error/1(y) -> Saturation/1
  Enable_Errors/1 -> Switch/2
  u/1 -> Switch/3, Sensor_Error/1(u)
  Add/1 -> Switch/1
  Sensor_Noise/1(noise) -> Add/2

== system Plant/Sensor_Model/Sensor_GPS/Bus_Constructor/GroundSpeed ==
  u_O_mPs : Inport
  v_O_mPs : Inport  Port=2
  Add : Sum
  Math Function : Math  Operator=square  SaturateOnIntegerOverflow=on
  Math Function1 : Math  Operator=square  SaturateOnIntegerOverflow=on
  Saturation : Saturate  UpperLimit=inf  LowerLimit=0
  Sqrt : Sqrt  SaturateOnIntegerOverflow=on
  gSpeed_mPs : Outport
  wires:
  Sqrt/1 -> gSpeed_mPs/1
  Math Function/1 -> Add/1
  Math Function1/1 -> Add/2
  Saturation/1 -> Sqrt/1
  Add/1 -> Saturation/1
  u_O_mPs/1 -> Math Function/1
  v_O_mPs/1 -> Math Function1/1

== system Plant/Sensor_Model/Sensor_GPS/Bus_Constructor/WGS84_Position ==
  pos_WGS84 : Inport
  Demux1 : Demux  Outputs=3
  Signal Conversion : SignalConversion  OverrideOpt=off
  Signal Conversion1 : SignalConversion  OverrideOpt=off
  Signal Conversion2 : SignalConversion  OverrideOpt=off
  lon : Outport
  lat : Outport  Port=2
  height : Outport  Port=3
  wires:
  Demux1/3 -> Signal Conversion2/1  "POS_h_WGS84"
  Signal Conversion/1 -> lon/1
  Demux1/1 -> Signal Conversion/1  "POS_lon_WGS84"
  pos_WGS84/1 -> Demux1/1
  Demux1/2 -> Signal Conversion1/1  "POS_lat_WGS84"
  Signal Conversion1/1 -> lat/1
  Signal Conversion2/1 -> height/1

== system Plant/Sensor_Model/Sensor_GPS/GPS/Bus_Constructor ==
  WGS84_pos_meas : Inport
  vel_O_meas : Inport  Port=2
  numSV : Inport  Port=3
  fixType : Inport  Port=4
  h_Acc_m : Inport  Port=5
  v_Acc_m : Inport  Port=6
  s_Acc_mDs : Inport  Port=7
  Bus Creator : BusCreator  Inputs=7
  GPS_Raw : Outport
  wires:
  WGS84_pos_meas/1 -> Bus Creator/1  "WGS84_pos"
  vel_O_meas/1 -> Bus Creator/2  "vel_O"
  numSV/1 -> Bus Creator/3  "numSV"
  fixType/1 -> Bus Creator/4  "fixType"
  h_Acc_m/1 -> Bus Creator/5  "hAcc"
  v_Acc_m/1 -> Bus Creator/6  "vAcc"
  s_Acc_mDs/1 -> Bus Creator/7  "sAcc"
  Bus Creator/1 -> GPS_Raw/1

== system Plant/Sensor_Model/Sensor_GPS/GPS/Physical_Model ==
  note: Transfer Delay
  States : Inport
  Bus Selector : BusSelector  OutputSignals=Plant_States.lon,Plant_States.lat,Plant_States.alt
  Bus Selector1 : BusSelector  OutputSignals=Plant_States.vel_x_O,Plant_States.vel_y_O,Plant_States.vel_z_O
  Delay : Delay  DelayLength=150/(PLANT_CONST.dt*1e3)
  Delay1 : Delay  DelayLength=100/(PLANT_CONST.dt*1e3)
  Vector Concatenate : Concatenate  NumInputs=3  Mode=Multidimensional array
  Vector Concatenate1 : Concatenate  NumInputs=3  Mode=Multidimensional array
  WGS84_pos_rad : Outport  Unit=rad/s
  vel_O_mPs : Outport  Port=2  Unit=m/s  PortDimensions=[3 1]
  wires:
  Bus Selector/3 -> Vector Concatenate/3  "<alt>"
  Bus Selector/2 -> Vector Concatenate/2  "<lat>"
  Bus Selector/1 -> Vector Concatenate/1  "<lon>"
  Vector Concatenate/1 -> Delay/1
  Bus Selector1/2 -> Vector Concatenate1/2  "<vel_y_O>"
  Bus Selector1/3 -> Vector Concatenate1/3  "<vel_z_O>"
  States/1 -> Bus Selector1/1, Bus Selector/1
  Vector Concatenate1/1 -> Delay1/1
  Bus Selector1/1 -> Vector Concatenate1/1  "<vel_x_O>"
  Delay/1 -> WGS84_pos_rad/1
  Delay1/1 -> vel_O_mPs/1

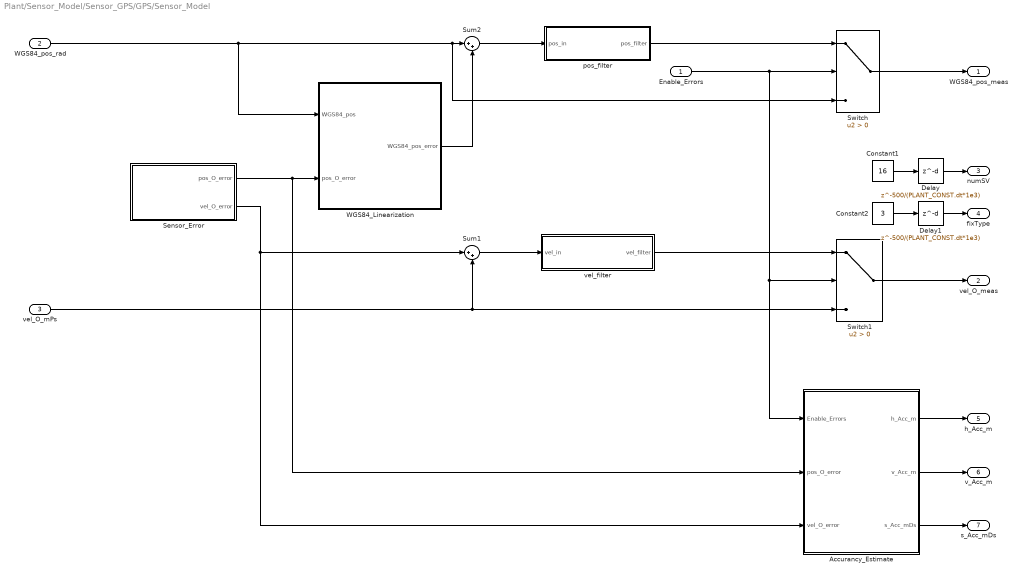
== system Plant/Sensor_Model/Sensor_GPS/GPS/Sensor_Model ==
  Enable_Errors : Inport
  WGS84_pos_rad : Inport  Port=2
  vel_O_mPs : Inport  Port=3
  Accurancy_Estimate : Subsystem
  Constant1 : Constant  Value=16  OutDataTypeStr=Inherit: Inherit via back propagation
  Constant2 : Constant  Value=3  OutDataTypeStr=Inherit: Inherit via back propagation
  Delay : Delay  DelayLength=500/(PLANT_CONST.dt*1e3)
  Delay1 : Delay  DelayLength=500/(PLANT_CONST.dt*1e3)
  Sensor_Error : Subsystem
  Sum1 : Sum  Inputs=|++
  Sum2 : Sum  Inputs=|++
  Switch : Switch  Criteria=u2 > Threshold
  Switch1 : Switch  Criteria=u2 > Threshold
  WGS84_Linearization : Subsystem
  pos_filter : Subsystem
  vel_filter : Subsystem
  WGS84_pos_meas : Outport
  vel_O_meas : Outport  Port=2
  numSV : Outport  Port=3
  fixType : Outport  Port=4
  h_Acc_m : Outport  Port=5
  v_Acc_m : Outport  Port=6
  s_Acc_mDs : Outport  Port=7
  wires:
  Constant2/1 -> Delay1/1
  Constant1/1 -> Delay/1
  Switch/1 -> WGS84_pos_meas/1
  Switch1/1 -> vel_O_meas/1
  Sum2/1 -> pos_filter/1(pos_in)
  Sensor_Error/1(pos_O_error) -> Accurancy_Estimate/2(pos_O_error), WGS84_Linearization/2(pos_O_error)
  Sum1/1 -> vel_filter/1(vel_in)
  Sensor_Error/2(vel_O_error) -> Accurancy_Estimate/3(vel_O_error), Sum1/1
  WGS84_Linearization/1(WGS84_pos_error) -> Sum2/2
  Accurancy_Estimate/1(h_Acc_m) -> h_Acc_m/1
  Accurancy_Estimate/3(s_Acc_mDs) -> s_Acc_mDs/1
  Accurancy_Estimate/2(v_Acc_m) -> v_Acc_m/1
  pos_filter/1(pos_filter) -> Switch/1
  WGS84_pos_rad/1 -> Switch/3, Sum2/1, WGS84_Linearization/1(WGS84_pos)
  vel_O_mPs/1 -> Switch1/3, Sum1/2
  vel_filter/1(vel_filter) -> Switch1/1
  Enable_Errors/1 -> Switch/2, Accurancy_Estimate/1(Enable_Errors), Switch1/2
  Delay/1 -> numSV/1
  Delay1/1 -> fixType/1

== system Plant/Sensor_Model/Sensor_IMU/Accelerometer/Bus_Constructor ==
  Output : Inport
  Bus Creator : BusCreator  Inputs=3
  Demux : Demux  Outputs=3
  Acc_Raw : Outport
  wires:
  Demux/2 -> Bus Creator/2  "Acc_y_mPs2"
  Demux/3 -> Bus Creator/3  "Acc_z_mPs2"
  Demux/1 -> Bus Creator/1  "Acc_x_mPs2"
  Bus Creator/1 -> Acc_Raw/1
  Output/1 -> Demux/1

== system Plant/Sensor_Model/Sensor_IMU/Accelerometer/Physical_Model ==
  States : Inport
  Enable_Errors : Inport  Port=2
  Sum : Sum  Inputs=|++
  Switch : Switch  Criteria=u2 > Threshold  OutDataTypeStr=single
  Vibration_Model : Subsystem  TreatAsAtomicUnit=on  mask{gain=Sensor_Model.Acc.Vibration.Gain}
      mask prompts: gain "Vibration gain"
      mask help: propeller vibration model
      settings: RTWSystemCode=Inline
  prop_vel : Subsystem
  specific_force : Subsystem
  sfor_B_mPs2 : Outport  Unit=m/s^2
  wires:
  States/1 -> specific_force/1(States), prop_vel/1(States)
  Switch/1 -> sfor_B_mPs2/1
  prop_vel/1(omega_radDs) -> Vibration_Model/1(prop_rot_radPs)
  specific_force/1(sfor_B_mPs2) -> Sum/2, Switch/3
  Enable_Errors/1 -> Switch/2
  Vibration_Model/1(vibration) -> Sum/1
  Sum/1 -> Switch/1

== system Plant/Sensor_Model/Sensor_IMU/Accelerometer/Sensor_Model ==
  Enable_Errors : Inport
  u : Inport  Port=2
  First Order LPF : FMT_Model_Lib/Filter/First Order LPF  fc=Sensor_Model.Acc.Cutoff_frequency_Hz
      settings: SourceProductName=FMT Toolbox
  Saturation : Saturate  UpperLimit=Sensor_Model.Acc.Upper_limit  LowerLimit=Sensor_Model.Acc.Lower_limit
  Sensor_Error : Subsystem
  Sensor_Noise : Subsystem
  Sum : Sum  Inputs=|++
  Switch : Switch  Criteria=u2 > Threshold
  y : Outport
  wires:
  Switch/1 -> y/1
  Saturation/1 -> Sum/1
  First Order LPF/1 -> Saturation/1
  Sensor_Error/1(y) -> First Order LPF/1
  Sensor_Noise/1(noise) -> Sum/2
  Enable_Errors/1 -> Switch/2
  u/1 -> Switch/3, Sensor_Error/1(u)
  Sum/1 -> Switch/1

== system Plant/Sensor_Model/Sensor_IMU/Gyroscope/Bus_Constructor ==
  Output : Inport
  Bus Creator : BusCreator  Inputs=3
  Demux : Demux  Outputs=3
  Gyro_Raw : Outport
  wires:
  Demux/1 -> Bus Creator/1  "Gyro_x_radPs"
  Demux/2 -> Bus Creator/2  "Gyro_y_radPs"
  Demux/3 -> Bus Creator/3  "Gyro_z_radPs"
  Bus Creator/1 -> Gyro_Raw/1
  Output/1 -> Demux/1

== system Plant/Sensor_Model/Sensor_IMU/Gyroscope/Physical_Model ==
  States : Inport
  Enable_Errors : Inport  Port=2
  Sum : Sum  Inputs=|++
  Switch : Switch  Criteria=u2 > Threshold
  Vibration_Model : Subsystem  TreatAsAtomicUnit=on  mask{gain=Sensor_Model.Gyro.Vibration.Gain}
      mask prompts: gain "Vibration gain"
      mask help: propeller vibration model
      settings: RTWSystemCode=Inline
  prop_vel : Subsystem
  rotation_speed : Subsystem
  gyr_B_radDs : Outport  Unit=rad/s
  wires:
  States/1 -> rotation_speed/1(States), prop_vel/1(States)
  Switch/1 -> gyr_B_radDs/1
  prop_vel/1(omega_radPs) -> Vibration_Model/1(prop_rot_radPs)
  rotation_speed/1(rot_radPs) -> Sum/2, Switch/3
  Enable_Errors/1 -> Switch/2
  Vibration_Model/1(vibration) -> Sum/1
  Sum/1 -> Switch/1

== system Plant/Sensor_Model/Sensor_IMU/Gyroscope/Sensor_Model ==
  Enable_Errors : Inport
  u : Inport  Port=2
  First Order LPF : FMT_Model_Lib/Filter/First Order LPF  fc=Sensor_Model.Gyro.Cutoff_frequency_Hz
      settings: SourceProductName=FMT Toolbox
  Saturation : Saturate  UpperLimit=Sensor_Model.Gyro.Range  LowerLimit=-Sensor_Model.Gyro.Range
  Sensor_Error : Subsystem
  Sensor_Noise : Subsystem
  Sum : Sum  Inputs=|++
  Switch : Switch  Criteria=u2 > Threshold
  y : Outport
  wires:
  Switch/1 -> y/1
  Saturation/1 -> Sum/1
  First Order LPF/1 -> Saturation/1
  Sensor_Error/1(y) -> First Order LPF/1
  Sensor_Noise/1(noise) -> Sum/2
  Enable_Errors/1 -> Switch/2
  u/1 -> Switch/3, Sensor_Error/1(u)
  Sum/1 -> Switch/1

== system Plant/Sensor_Model/Sensor_MAG/Magnetometer/Bus_Constructor ==
  Output : Inport
  Bus Creator : BusCreator  Inputs=3
  Demux : Demux  Outputs=3
  Mag_Raw : Outport
  wires:
  Demux/2 -> Bus Creator/2  "Mag_y_gauss"
  Demux/1 -> Bus Creator/1  "Mag_x_gauss"
  Bus Creator/1 -> Mag_Raw/1
  Demux/3 -> Bus Creator/3  "Mag_z_gauss"
  Output/1 -> Demux/1
